simulink model "kuksa_v2_demo"  (R2026b)
settings: Solver=VariableStepAuto  StopTime=inf
settings Model: DataDictionary=kuksa_v2_demo.sldd  Creator=SET6KOR  LastModifiedBy=SET6KOR
settings DataIOCC: SaveOutput=off  SaveTime=off  SignalLogging=off

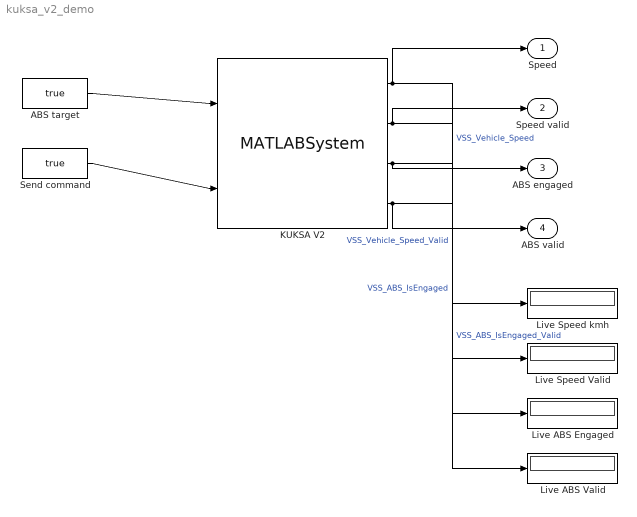
== system kuksa_v2_demo ==
  ABS target : Constant  Value=true  OutDataTypeStr=boolean
  KUKSA V2 : MATLABSystem  System=KuksaV2System  Host=127.0.0.1  Port=55556  Timeout=3  SampleTime=0.1  EnableActuation=true  AllowInsecureRemote=false
      mask Type: KuksaV2System
  Live ABS Engaged : Display
  Live ABS Valid : Display
  Live Speed Valid : Display
  Live Speed kmh : Display
  Send command : Constant  Value=true  OutDataTypeStr=boolean
  Speed : Outport
  Speed valid : Outport  Port=2
  ABS engaged : Outport  Port=3
  ABS valid : Outport  Port=4
  wires:
  ABS target/1 -> KUKSA V2/1
  Send command/1 -> KUKSA V2/2
  KUKSA V2/1 -> Speed/1, Live Speed kmh/1  "VSS_Vehicle_Speed"
  KUKSA V2/2 -> Speed valid/1, Live Speed Valid/1  "VSS_Vehicle_Speed_Valid"
  KUKSA V2/3 -> ABS engaged/1, Live ABS Engaged/1  "VSS_ABS_IsEngaged"
  KUKSA V2/4 -> ABS valid/1, Live ABS Valid/1  "VSS_ABS_IsEngaged_Valid"
